simulink model "course_lab5_frequency_inertia"  (R2024b)
settings: Solver=ode45  StartTime=0.0  StopTime=0.1  MaxStep=6.666666666666667e-05  RelTol=1e-7  AbsTol=1e-9
model workspace (MAT data in the model file):
  A = 1
  GBW = 1000000
  K = 1
  T = 0.001
  den = [0.001 1]
  frequency = 100
  num = [0 1]
  web_input = timeseries
  web_input.Name = 'unnamed'
  web_input.DataInfo = tsdata.datametadata
  web_input.DataInfo.Interpolation = tsdata.interpolation
  web_input.DataInfo.Interpolation.Fhandle : function handle (value not decoded)
  web_input.DataInfo.Interpolation.Name = 'linear'
  web_input.TimeInfo = tsdata.timemetadata
  web_input.TimeInfo.Length = 1501
  web_input.TimeInfo.DuplicateTimes = 0
  web_input.TimeInfo.Time_ = [0 6.66666666667e-05 0.000133333333333 0.0002 0.000266666666667 0.000333333333333 0.0004 0.000466666666667 0.000533333333333 0.0006 0.000666666666667 0.000733333333333 ... (1501 elements, 1501x1)]
  web_input.TimeInfo.Initialized = 1
  web_input.QualityInfo = tsdata.qualmetadata
  web_input.Data_ = [0 0.0418756537292 0.0836778433323 0.125333233564 0.166768746716 0.207911690818 0.248689887165 0.289031796944 0.328866646739 0.368124552685 0.406736643076 0.444635179185 ... (1501 elements, 1501x1)]
  wn = 22.36068
  zeta = 0.223607
settings Model: Creator=33657  LastModifiedBy=33657

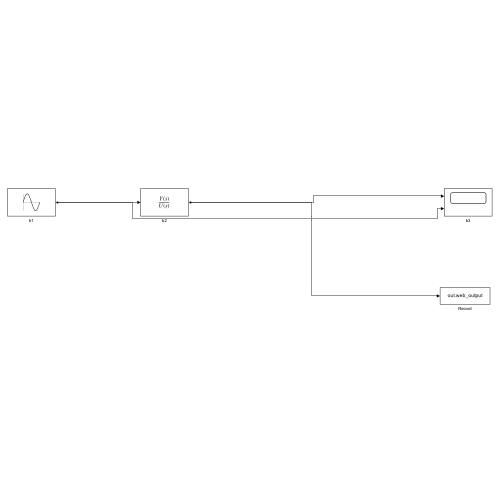
[thumbnail: Simulink's stored preview of the top-level diagram]
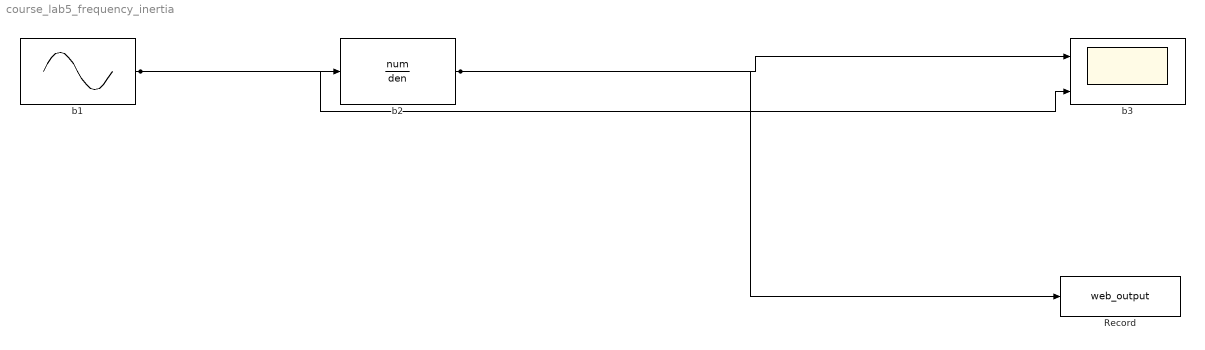
== system course_lab5_frequency_inertia ==
  Record : ToWorkspace  VariableName=web_output  SaveFormat=Timeseries  SampleTime=-1
  b1 : Sin  Amplitude=A  Frequency=2*pi*frequency  SampleTime=0
  b2 : TransferFcn  Numerator=num  Denominator=den
  b3 : Scope  NumInputPorts=2
  wires:
  b1/1 -> b2/1, b3/2
  b2/1 -> b3/1, Record/1
